simulink model "fft_test"  (Simulink 7.4)
settings: Solver=VariableStepDiscrete  StartTime=0.0  StopTime=500  RelTol=1e-3
libraries: xbsIndex_r4 x1178, casper_library_misc x68, casper_library_delays x13, casper_library_reorder x4, casper_library_ffts_twiddle x2
(part 7 of 11)

== system fft_test/fft/fft_direct/butterfly2_1/twiddle ==
  a : Inport
  b : Inport  Port=2
  sync : Inport  Port=3
  AddSub : xbsIndex_r4/AddSub  mode=Subtraction  use_carryin=off  use_carryout=off  en=off  latency=add_latency  precision=Full  arith_type=Unsigned  n_bits=16  bin_pt=14  quantization=Truncate  overflow=Wrap  dbl_ovrd=off  use_behavioral_HDL=on  hw_selection=Fabric  pipelined=off  block_type=addsub
  AddSub1 : xbsIndex_r4/AddSub  mode=Addition  use_carryin=off  use_carryout=off  en=off  latency=add_latency  precision=Full  arith_type=Unsigned  n_bits=16  bin_pt=14  quantization=Truncate  overflow=Wrap  dbl_ovrd=off  use_behavioral_HDL=on  hw_selection=Fabric  pipelined=off  block_type=addsub
  AddSub2 : xbsIndex_r4/AddSub  mode=Addition  use_carryin=off  use_carryout=off  en=off  latency=add_latency  precision=Full  arith_type=Unsigned  n_bits=16  bin_pt=14  quantization=Truncate  overflow=Wrap  dbl_ovrd=off  use_behavioral_HDL=on  hw_selection=Fabric  pipelined=off  block_type=addsub
  AddSub3 : xbsIndex_r4/AddSub  mode=Subtraction  use_carryin=off  use_carryout=off  en=off  latency=add_latency  precision=Full  arith_type=Unsigned  n_bits=16  bin_pt=14  quantization=Truncate  overflow=Wrap  dbl_ovrd=off  use_behavioral_HDL=on  hw_selection=Fabric  pipelined=off  block_type=addsub
  AddSub4 : xbsIndex_r4/AddSub  mode=Addition  use_carryin=off  use_carryout=off  en=off  latency=add_latency  precision=Full  arith_type=Unsigned  n_bits=16  bin_pt=14  quantization=Truncate  overflow=Wrap  dbl_ovrd=off  use_behavioral_HDL=on  hw_selection=Fabric  pipelined=off  block_type=addsub
  c_to_ri1 : casper_library_misc/c_to_ri  SystemSampleTime=-1  n_bits=8  bin_pt=7
      settings: AttributesFormatString=8_7 r/i
  c_to_ri2 : casper_library_misc/c_to_ri  SystemSampleTime=-1  n_bits=7  bin_pt=5
      settings: AttributesFormatString=7_5 r/i
  c_to_ri3 : casper_library_misc/c_to_ri  SystemSampleTime=-1  n_bits=input_bit_width  bin_pt=input_bit_width-1
      settings: AttributesFormatString=8_7 r/i
  coeff_gen : Subsystem  AncestorBlock=casper_library_ffts_twiddle_coeff_gen/coeff_gen  mask(coeff_gen){Coeffs=getfield( getfield( get_param( gcb,'UserData' ), 'parameters'),'Coeffs'), coeff_bit_width=7, StepPeriod=0, bram_latency=1, coeffs_bram=off}
      mask prompts: Coeffs "Coefficients: (0 to 2^(FFTSize-1)-1)"; coeff_bit_width "Coefficient Bit Width:"; StepPeriod "Step Period: (2^?)"; bram_latency "Latency:"; coeffs_bram "Store coefficients in BRAM"
      mask help: Generates a sequence of complex coefficients
      mask init:
      | coeff_gen_init( gcb, ...
      |     'Coeffs', Coeffs, ...
      |     'coeff_bit_width', coeff_bit_width, ...
      |     'StepPeriod', StepPeriod, ...
      |     'bram_latency', bram_latency, ...
      |     'coeffs_bram', coeffs_bram);
      settings: AttributesFormatString=16 @ (7,5)
      mask CallbackString:
      | Coeffs = eval(get_param(gcb, 'Coeffs'));
      | if( length(Coeffs) == 1 ),
      |     set_param(gcb, 'MaskVisibilities',{'on','on','off','off','off'});
      | else
      |     set_param(gcb, 'MaskVisibilities',{'on','on','on','on','on'});
      | end||||
  convert2 : xbsIndex_r4/Convert  arith_type="Signed  (2's comp)"  n_bits=input_bit_width+5  bin_pt=input_bit_width+1  quantization="Round  (unbiased: +/- Inf)"  overflow=Saturate  latency=conv_latency  dbl_ovrd=off  pipeline=on  block_type=convert
      settings: block_version=11.4
  convert3 : xbsIndex_r4/Convert  arith_type="Signed  (2's comp)"  n_bits=input_bit_width+5  bin_pt=input_bit_width+1  quantization="Round  (unbiased: +/- Inf)"  overflow=Saturate  latency=conv_latency  dbl_ovrd=off  pipeline=on  block_type=convert
      settings: block_version=11.4
  delay0 : xbsIndex_r4/Delay  en=off  latency=mult_latency + 2*add_latency + bram_latency + conv_latency  dbl_ovrd=off  reg_retiming=off  block_type=delay
      settings: block_version=11.4
  delay1 : xbsIndex_r4/Delay  en=off  latency=bram_latency  dbl_ovrd=off  reg_retiming=off  block_type=delay
      settings: block_version=11.4
  delay2 : xbsIndex_r4/Delay  en=off  latency=mult_latency + 2*add_latency + bram_latency + conv_latency  dbl_ovrd=off  reg_retiming=off  block_type=delay
      settings: block_version=11.4
  delay3 : xbsIndex_r4/Delay  en=off  latency=add_latency  dbl_ovrd=off  reg_retiming=on  block_type=delay
      settings: block_version=11.4
  delay4 : xbsIndex_r4/Delay  en=off  latency=add_latency  dbl_ovrd=off  reg_retiming=on  block_type=delay
      settings: block_version=11.4
  delay5 : xbsIndex_r4/Delay  en=off  latency=add_latency  dbl_ovrd=off  reg_retiming=on  block_type=delay
      settings: block_version=11.4
  mult0 : xbsIndex_r4/Mult  precision=Full  arith_type="Signed  (2's comp)"  n_bits=16  bin_pt=14  quantization=Truncate  overflow=Wrap  en=off  latency=mult_latency  dbl_ovrd=off  use_behavioral_HDL=on  opt=Speed  use_embedded=off  optimum_pipeline=off  pipeline=on  use_rpm=on  placement_style=Triangular  block_type=mult
      settings: block_version=11.4
  mult1 : xbsIndex_r4/Mult  precision=Full  arith_type="Signed  (2's comp)"  n_bits=16  bin_pt=14  quantization=Truncate  overflow=Wrap  en=off  latency=mult_latency  dbl_ovrd=off  use_behavioral_HDL=on  opt=Speed  use_embedded=off  optimum_pipeline=off  pipeline=on  use_rpm=on  placement_style=Triangular  block_type=mult
      settings: block_version=11.4
  mult2 : xbsIndex_r4/Mult  precision=Full  arith_type="Signed  (2's comp)"  n_bits=16  bin_pt=14  quantization=Truncate  overflow=Wrap  en=off  latency=mult_latency  dbl_ovrd=off  use_behavioral_HDL=on  opt=Speed  use_embedded=off  optimum_pipeline=off  pipeline=on  use_rpm=on  placement_style=Triangular  block_type=mult
      settings: block_version=11.4
  a_re : Outport
  a_im : Outport  Port=2
  bw_re : Outport  Port=3
  bw_im : Outport  Port=4
  sync_out : Outport  Port=5
  wires:
  a/1 -> delay0/1
  delay0/1 -> c_to_ri1/1
  c_to_ri1/1 -> a_re/1
  c_to_ri1/2 -> a_im/1
  sync/1 -> delay2/1, coeff_gen/1(rst)
  delay2/1 -> sync_out/1
  coeff_gen/1(w) -> c_to_ri2/1
  c_to_ri2/1 -> AddSub2/1, AddSub3/2, delay5/1
  c_to_ri2/2 -> AddSub2/2, AddSub3/1
  b/1 -> delay1/1
  delay1/1 -> c_to_ri3/1
  c_to_ri3/1 -> AddSub1/1, delay3/1
  c_to_ri3/2 -> AddSub1/2, delay4/1
  AddSub1/1 -> mult0/1
  delay5/1 -> mult0/2
  delay4/1 -> mult1/1
  AddSub2/1 -> mult1/2
  delay3/1 -> mult2/1
  AddSub3/1 -> mult2/2
  mult0/1 -> AddSub/1, AddSub4/1
  mult1/1 -> AddSub/2
  mult2/1 -> AddSub4/2
  AddSub/1 -> convert2/1
  convert2/1 -> bw_re/1
  AddSub4/1 -> convert3/1
  convert3/1 -> bw_im/1

== system fft_test/fft/fft_unscrambler/square_transposer/barrel_switcher ==
  sel : Inport  OutDataType=sfix(16)  OutScaling=2^0
  sync_in : Inport  Port=2  OutDataType=sfix(16)  OutScaling=2^0
  In1 : Inport  Port=3  OutDataType=sfix(16)  OutScaling=2^0
  In2 : Inport  Port=4  OutDataType=sfix(16)  OutScaling=2^0
  In3 : Inport  Port=5
  In4 : Inport  Port=6
  Delay1 : xbsIndex_r4/Delay  en=off  latency=1  dbl_ovrd=off  reg_retiming=off  block_type=delay
      settings: block_version=10.1.1
  Delay_sync : xbsIndex_r4/Delay  en=off  latency=2  dbl_ovrd=off  reg_retiming=off  block_type=delay
      settings: xl_area=[0, 0, 0, 0, 0, 0, 0]  block_version=9.1.01
  Mux11 : xbsIndex_r4/Mux  inputs=2  en=off  latency=1  precision=Full  arith_type="Signed  (2's comp)"  n_bits=8  bin_pt=2  quantization=Truncate  overflow=Wrap  dbl_ovrd=off  block_type=mux
      settings: xl_area=[0, 0, 0, 0, 0, 0, 0]  block_version=9.1.01
  Mux{12,22,31..32,41..42} (6 alike) : xbsIndex_r4/Mux  inputs=2  en=off  latency=1  precision=Full  arith_type=Unsigned  n_bits=16  bin_pt=14  quantization=Truncate  overflow=Wrap  dbl_ovrd=off  block_type=mux
      settings: block_version=10.1.1
  Mux21 : xbsIndex_r4/Mux  inputs=2  en=off  latency=1  precision=Full  arith_type="Signed  (2's comp)"  n_bits=8  bin_pt=2  quantization=Truncate  overflow=Wrap  dbl_ovrd=off  block_type=mux
      settings: xl_area=[0, 0, 0, 0, 0, 0, 0]  block_version=9.1.01
  Slice1 : xbsIndex_r4/Slice  nbits=1  boolean_output=off  mode=Upper Bit Location + Width  bit1=-0  base1=MSB of Input  bit0=0  base0=LSB of Input  dbl_ovrd=off  block_type=slice
      settings: infoedit="Extracts a given range of bits from each input sample and presents it at the output.  The output type is ordinarily unsigned with binary point at zero, but can be Boolean when the slice is one bit wide.<P><P>Hardware notes: In hardware this block costs nothing."  block_version=9.1.01
  Slice2 : xbsIndex_r4/Slice  nbits=1  boolean_output=off  mode=Upper Bit Location + Width  bit1=-1  base1=MSB of Input  bit0=0  base0=LSB of Input  dbl_ovrd=off  block_type=slice
      settings: infoedit="Extracts a given range of bits from each input sample and presents it at the output.  The output type is ordinarily unsigned with binary point at zero, but can be Boolean when the slice is one bit wide.<P><P>Hardware notes: In hardware this block costs nothing."  block_version=10.1.1
  sync_out : Outport  OutDataType=sfix(16)  OutScaling=2^0
  Out1 : Outport  Port=2  OutDataType=sfix(16)  OutScaling=2^0
  Out2 : Outport  Port=3  OutDataType=sfix(16)  OutScaling=2^0
  Out3 : Outport  Port=4
  Out4 : Outport  Port=5
  wires:
  sync_in/1 -> Delay_sync/1
  Delay_sync/1 -> sync_out/1
  sel/1 -> Slice1/1, Delay1/1
  Delay1/1 -> Slice2/1
  Slice1/1 -> Mux11/1, Mux21/1, Mux31/1, Mux41/1
  Slice2/1 -> Mux12/1, Mux22/1, Mux32/1, Mux42/1
  In1/1 -> Mux11/2, Mux31/3
  Mux12/1 -> Out1/1
  In2/1 -> Mux21/2, Mux41/3
  Mux22/1 -> Out2/1
  In3/1 -> Mux31/2, Mux11/3
  Mux32/1 -> Out3/1
  In4/1 -> Mux41/2, Mux21/3
  Mux42/1 -> Out4/1
  Mux11/1 -> Mux12/2, Mux42/3
  Mux21/1 -> Mux22/2, Mux12/3
  Mux31/1 -> Mux32/2, Mux22/3
  Mux41/1 -> Mux42/2, Mux32/3

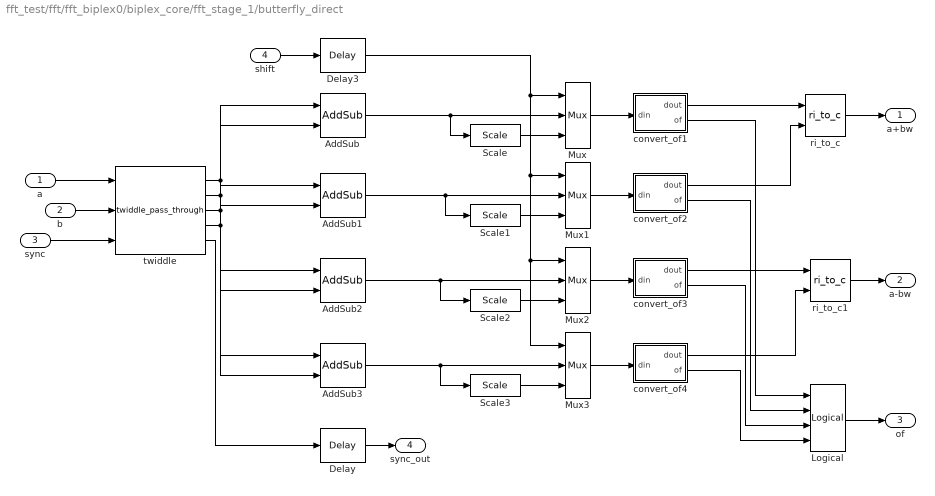
== system fft_test/fft/fft_biplex0/biplex_core/fft_stage_1/butterfly_direct ==
  a : Inport  OutDataType=sfix(16)  OutScaling=2^0
  b : Inport  Port=2  OutDataType=sfix(16)  OutScaling=2^0
  sync : Inport  Port=3  OutDataType=sfix(16)  OutScaling=2^0
  shift : Inport  Port=4  OutDataType=sfix(16)  OutScaling=2^0
  AddSub : xbsIndex_r4/AddSub  mode=Addition  use_carryin=off  use_carryout=off  en=off  latency=add_latency  precision=Full  arith_type=Unsigned  n_bits=8  bin_pt=2  quantization=Truncate  overflow=Wrap  dbl_ovrd=off  use_behavioral_HDL=off  hw_selection=DSP48  pipelined=on  use_rpm=on  block_type=addsub
      settings: xl_area=[0, 0, 0, 0, 0, 0, 0]  block_version=9.1.01
  AddSub1 : xbsIndex_r4/AddSub  mode=Addition  use_carryin=off  use_carryout=off  en=off  latency=add_latency  precision=Full  arith_type=Unsigned  n_bits=8  bin_pt=2  quantization=Truncate  overflow=Wrap  dbl_ovrd=off  use_behavioral_HDL=off  hw_selection=DSP48  pipelined=on  use_rpm=on  block_type=addsub
      settings: xl_area=[0, 0, 0, 0, 0, 0, 0]  block_version=9.1.01
  AddSub2 : xbsIndex_r4/AddSub  mode=Subtraction  use_carryin=off  use_carryout=off  en=off  latency=add_latency  precision=Full  arith_type=Unsigned  n_bits=8  bin_pt=2  quantization=Truncate  overflow=Wrap  dbl_ovrd=off  use_behavioral_HDL=off  hw_selection=DSP48  pipelined=on  use_rpm=on  block_type=addsub
      settings: xl_area=[0, 0, 0, 0, 0, 0, 0]  block_version=9.1.01
  AddSub3 : xbsIndex_r4/AddSub  mode=Subtraction  use_carryin=off  use_carryout=off  en=off  latency=add_latency  precision=Full  arith_type=Unsigned  n_bits=8  bin_pt=2  quantization=Truncate  overflow=Wrap  dbl_ovrd=off  use_behavioral_HDL=off  hw_selection=DSP48  pipelined=on  use_rpm=on  block_type=addsub
      settings: xl_area=[0, 0, 0, 0, 0, 0, 0]  block_version=9.1.01
  Delay : xbsIndex_r4/Delay  en=off  latency=add_latency + conv_latency + 1  dbl_ovrd=off  reg_retiming=on  block_type=delay
      settings: xl_area=[0, 0, 0, 0, 0, 0, 0]  block_version=9.1.01
  Delay3 : xbsIndex_r4/Delay  en=off  latency=add_latency  dbl_ovrd=off  reg_retiming=off  block_type=delay
      settings: xl_area=[0, 0, 0, 0, 0, 0, 0]  block_version=9.1.01
  Logical : xbsIndex_r4/Logical  logical_function=OR  inputs=4  en=off  latency=0  precision=Full  arith_type=Unsigned  n_bits=16  bin_pt=0  align_bp=on  dbl_ovrd=off  block_type=logical
      settings: block_version=10.1.1
  Mux{,1..3} (4 alike) : xbsIndex_r4/Mux  inputs=2  en=off  latency=1  precision=Full  arith_type="Signed  (2's comp)"  n_bits=8  bin_pt=2  quantization=Truncate  overflow=Wrap  dbl_ovrd=off  block_type=mux
      settings: xl_area=[0, 0, 0, 0, 0, 0, 0]  block_version=9.1.01
  Scale{,1..3} (4 alike) : xbsIndex_r4/Scale  scale_factor=-1  dbl_ovrd=off  block_type=scale
      settings: infoedit=Scales input by a power of two by adjusting the binary point position.<P><P>Hardware notes: In hardware this block costs nothing.  block_version=9.1.01
  convert_of1 : Subsystem  AncestorBlock=casper_library_misc/convert_of  mask(convert_of){bit_width_i=10, binary_point_i=8, bit_width_o=8, binary_point_o=7, latency=2, overflow=Saturate, quantization=Round  (unbiased: +/- Inf)}
      mask prompts: bit_width_i "Bit Width In"; binary_point_i "Binary Point In"; bit_width_o "Bit Width Out"; binary_point_o "Binary Point Out"; overflow "Overflow Behaviour"; quantization "Quantization Behaviour"
      mask help:
      | Converts from one 2's complement bit-width
      | and/or binary point position to another.
      | Includes underflow/overflow indicator.
      mask init: same as fft_test/fft/fft_direct/butterfly1_0/convert_of1
      settings: AttributesFormatString=[10,8]->[8,7]
      mask StyleString: edit,edit,edit,edit,edit,popup(Wrap|Saturate|Error),popup(Truncate|Round  (unbiased: +/- Inf)|Round  (unbiased: even values))
  convert_of2 : Subsystem  AncestorBlock=casper_library_misc/convert_of  mask(convert_of){bit_width_i=10, binary_point_i=8, bit_width_o=8, binary_point_o=7, latency=2, overflow=Saturate, quantization=Round  (unbiased: +/- Inf)}
      mask prompts: bit_width_i "Bit Width In"; binary_point_i "Binary Point In"; bit_width_o "Bit Width Out"; binary_point_o "Binary Point Out"; overflow "Overflow Behaviour"; quantization "Quantization Behaviour"
      mask help:
      | Converts from one 2's complement bit-width
      | and/or binary point position to another.
      | Includes underflow/overflow indicator.
      mask init: same as fft_test/fft/fft_direct/butterfly1_0/convert_of1
      settings: AttributesFormatString=[10,8]->[8,7]
      mask StyleString: edit,edit,edit,edit,edit,popup(Wrap|Saturate|Error),popup(Truncate|Round  (unbiased: +/- Inf)|Round  (unbiased: even values))
  convert_of3 : Subsystem  AncestorBlock=casper_library_misc/convert_of  mask(convert_of){bit_width_i=10, binary_point_i=8, bit_width_o=8, binary_point_o=7, latency=2, overflow=Saturate, quantization=Round  (unbiased: +/- Inf)}
      mask prompts: bit_width_i "Bit Width In"; binary_point_i "Binary Point In"; bit_width_o "Bit Width Out"; binary_point_o "Binary Point Out"; overflow "Overflow Behaviour"; quantization "Quantization Behaviour"
      mask help:
      | Converts from one 2's complement bit-width
      | and/or binary point position to another.
      | Includes underflow/overflow indicator.
      mask init: same as fft_test/fft/fft_direct/butterfly1_0/convert_of1
      settings: AttributesFormatString=[10,8]->[8,7]
      mask StyleString: edit,edit,edit,edit,edit,popup(Wrap|Saturate|Error),popup(Truncate|Round  (unbiased: +/- Inf)|Round  (unbiased: even values))
  convert_of4 : Subsystem  AncestorBlock=casper_library_misc/convert_of  mask(convert_of){bit_width_i=10, binary_point_i=8, bit_width_o=8, binary_point_o=7, latency=2, overflow=Saturate, quantization=Round  (unbiased: +/- Inf)}
      mask prompts: bit_width_i "Bit Width In"; binary_point_i "Binary Point In"; bit_width_o "Bit Width Out"; binary_point_o "Binary Point Out"; overflow "Overflow Behaviour"; quantization "Quantization Behaviour"
      mask help:
      | Converts from one 2's complement bit-width
      | and/or binary point position to another.
      | Includes underflow/overflow indicator.
      mask init: same as fft_test/fft/fft_direct/butterfly1_0/convert_of1
      settings: AttributesFormatString=[10,8]->[8,7]
      mask StyleString: edit,edit,edit,edit,edit,popup(Wrap|Saturate|Error),popup(Truncate|Round  (unbiased: +/- Inf)|Round  (unbiased: even values))
  ri_to_c : casper_library_misc/ri_to_c  SystemSampleTime=-1
  ri_to_c1 : casper_library_misc/ri_to_c  SystemSampleTime=-1
  twiddle : casper_library_ffts_twiddle/twiddle_pass_through  SystemSampleTime=-1  FFTSize=4  input_bit_width=8  add_latency=2  mult_latency=3  bram_latency=1  conv_latency=2  opt_target=multipliers
  a+bw : Outport  OutDataType=sfix(16)  OutScaling=2^0
  a-bw : Outport  Port=2  OutDataType=sfix(16)  OutScaling=2^0
  of : Outport  Port=3  OutDataType=sfix(16)  OutScaling=2^0
  sync_out : Outport  Port=4  OutDataType=sfix(16)  OutScaling=2^0
  wires:
  convert_of4/2(of) -> Logical/4
  convert_of3/2(of) -> Logical/3
  convert_of2/2(of) -> Logical/2
  convert_of1/2(of) -> Logical/1
  convert_of4/1(dout) -> ri_to_c1/2
  Mux3/1 -> convert_of4/1(din)
  AddSub3/1 -> Scale3/1, Mux3/2
  Scale3/1 -> Mux3/3
  convert_of3/1(dout) -> ri_to_c1/1
  Mux2/1 -> convert_of3/1(din)
  AddSub2/1 -> Scale2/1, Mux2/2
  Scale2/1 -> Mux2/3
  convert_of2/1(dout) -> ri_to_c/2
  Mux1/1 -> convert_of2/1(din)
  AddSub1/1 -> Scale1/1, Mux1/2
  Scale1/1 -> Mux1/3
  convert_of1/1(dout) -> ri_to_c/1
  Mux/1 -> convert_of1/1(din)
  twiddle/4 -> AddSub3/2, AddSub1/2
  twiddle/3 -> AddSub2/2, AddSub/2
  twiddle/2 -> AddSub3/1, AddSub1/1
  twiddle/1 -> AddSub2/1, AddSub/1
  sync/1 -> twiddle/3
  b/1 -> twiddle/2
  a/1 -> twiddle/1
  ri_to_c/1 -> a+bw/1
  ri_to_c1/1 -> a-bw/1
  Delay/1 -> sync_out/1
  AddSub/1 -> Mux/2, Scale/1
  shift/1 -> Delay3/1
  Scale/1 -> Mux/3
  Delay3/1 -> Mux3/1, Mux2/1, Mux1/1, Mux/1
  Logical/1 -> of/1
  twiddle/5 -> Delay/1

== system fft_test/fft/fft_biplex0/biplex_core/fft_stage_1/delay_b ==
  In1 : Inport  OutDataType=sfix(16)  OutScaling=2^0
  delay_slr : xbsIndex_r4/Delay  en=off  latency=DelayLen  dbl_ovrd=off  reg_retiming=off  block_type=delay
      settings: xl_area=[0, 0, 0, 0, 0, 0, 0]  block_version=9.1.01
  Out1 : Outport  OutDataType=sfix(16)  OutScaling=2^0
  wires:
  delay_slr/1 -> Out1/1
  In1/1 -> delay_slr/1

== system fft_test/fft/fft_biplex0/biplex_core/fft_stage_1/delay_f ==
  In1 : Inport  OutDataType=sfix(16)  OutScaling=2^0
  delay_slr : xbsIndex_r4/Delay  en=off  latency=DelayLen  dbl_ovrd=off  reg_retiming=off  block_type=delay
      settings: xl_area=[0, 0, 0, 0, 0, 0, 0]  block_version=9.1.01
  Out1 : Outport  OutDataType=sfix(16)  OutScaling=2^0
  wires:
  delay_slr/1 -> Out1/1
  In1/1 -> delay_slr/1

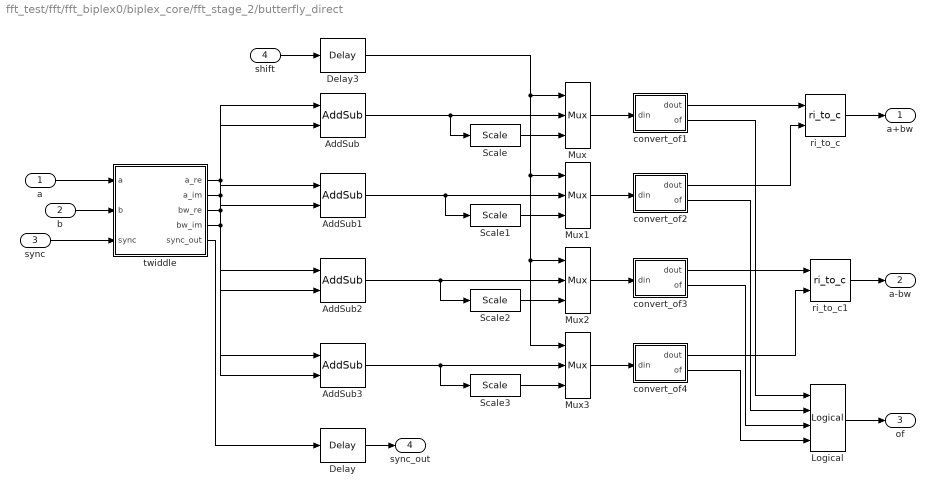
== system fft_test/fft/fft_biplex0/biplex_core/fft_stage_2/butterfly_direct ==
  a : Inport  OutDataType=sfix(16)  OutScaling=2^0
  b : Inport  Port=2  OutDataType=sfix(16)  OutScaling=2^0
  sync : Inport  Port=3  OutDataType=sfix(16)  OutScaling=2^0
  shift : Inport  Port=4  OutDataType=sfix(16)  OutScaling=2^0
  AddSub : xbsIndex_r4/AddSub  mode=Addition  use_carryin=off  use_carryout=off  en=off  latency=add_latency  precision=Full  arith_type=Unsigned  n_bits=8  bin_pt=2  quantization=Truncate  overflow=Wrap  dbl_ovrd=off  use_behavioral_HDL=off  hw_selection=DSP48  pipelined=on  use_rpm=on  block_type=addsub
      settings: xl_area=[0, 0, 0, 0, 0, 0, 0]  block_version=9.1.01
  AddSub1 : xbsIndex_r4/AddSub  mode=Addition  use_carryin=off  use_carryout=off  en=off  latency=add_latency  precision=Full  arith_type=Unsigned  n_bits=8  bin_pt=2  quantization=Truncate  overflow=Wrap  dbl_ovrd=off  use_behavioral_HDL=off  hw_selection=DSP48  pipelined=on  use_rpm=on  block_type=addsub
      settings: xl_area=[0, 0, 0, 0, 0, 0, 0]  block_version=9.1.01
  AddSub2 : xbsIndex_r4/AddSub  mode=Subtraction  use_carryin=off  use_carryout=off  en=off  latency=add_latency  precision=Full  arith_type=Unsigned  n_bits=8  bin_pt=2  quantization=Truncate  overflow=Wrap  dbl_ovrd=off  use_behavioral_HDL=off  hw_selection=DSP48  pipelined=on  use_rpm=on  block_type=addsub
      settings: xl_area=[0, 0, 0, 0, 0, 0, 0]  block_version=9.1.01
  AddSub3 : xbsIndex_r4/AddSub  mode=Subtraction  use_carryin=off  use_carryout=off  en=off  latency=add_latency  precision=Full  arith_type=Unsigned  n_bits=8  bin_pt=2  quantization=Truncate  overflow=Wrap  dbl_ovrd=off  use_behavioral_HDL=off  hw_selection=DSP48  pipelined=on  use_rpm=on  block_type=addsub
      settings: xl_area=[0, 0, 0, 0, 0, 0, 0]  block_version=9.1.01
  Delay : xbsIndex_r4/Delay  en=off  latency=add_latency + conv_latency + 1  dbl_ovrd=off  reg_retiming=on  block_type=delay
      settings: xl_area=[0, 0, 0, 0, 0, 0, 0]  block_version=9.1.01
  Delay3 : xbsIndex_r4/Delay  en=off  latency=add_latency  dbl_ovrd=off  reg_retiming=off  block_type=delay
      settings: xl_area=[0, 0, 0, 0, 0, 0, 0]  block_version=9.1.01
  Logical : xbsIndex_r4/Logical  logical_function=OR  inputs=4  en=off  latency=0  precision=Full  arith_type=Unsigned  n_bits=16  bin_pt=0  align_bp=on  dbl_ovrd=off  block_type=logical
      settings: block_version=10.1.1
  Mux{,1..3} (4 alike) : xbsIndex_r4/Mux  inputs=2  en=off  latency=1  precision=Full  arith_type="Signed  (2's comp)"  n_bits=8  bin_pt=2  quantization=Truncate  overflow=Wrap  dbl_ovrd=off  block_type=mux
      settings: xl_area=[0, 0, 0, 0, 0, 0, 0]  block_version=9.1.01
  Scale{,1..3} (4 alike) : xbsIndex_r4/Scale  scale_factor=-1  dbl_ovrd=off  block_type=scale
      settings: infoedit=Scales input by a power of two by adjusting the binary point position.<P><P>Hardware notes: In hardware this block costs nothing.  block_version=9.1.01
  convert_of1 : Subsystem  AncestorBlock=casper_library_misc/convert_of  mask(convert_of){bit_width_i=10, binary_point_i=8, bit_width_o=8, binary_point_o=7, latency=2, overflow=Saturate, quantization=Round  (unbiased: +/- Inf)}
      mask prompts: bit_width_i "Bit Width In"; binary_point_i "Binary Point In"; bit_width_o "Bit Width Out"; binary_point_o "Binary Point Out"; overflow "Overflow Behaviour"; quantization "Quantization Behaviour"
      mask help:
      | Converts from one 2's complement bit-width
      | and/or binary point position to another.
      | Includes underflow/overflow indicator.
      mask init: same as fft_test/fft/fft_direct/butterfly1_0/convert_of1
      settings: AttributesFormatString=[10,8]->[8,7]
      mask StyleString: edit,edit,edit,edit,edit,popup(Wrap|Saturate|Error),popup(Truncate|Round  (unbiased: +/- Inf)|Round  (unbiased: even values))
  convert_of2 : Subsystem  AncestorBlock=casper_library_misc/convert_of  mask(convert_of){bit_width_i=10, binary_point_i=8, bit_width_o=8, binary_point_o=7, latency=2, overflow=Saturate, quantization=Round  (unbiased: +/- Inf)}
      mask prompts: bit_width_i "Bit Width In"; binary_point_i "Binary Point In"; bit_width_o "Bit Width Out"; binary_point_o "Binary Point Out"; overflow "Overflow Behaviour"; quantization "Quantization Behaviour"
      mask help:
      | Converts from one 2's complement bit-width
      | and/or binary point position to another.
      | Includes underflow/overflow indicator.
      mask init: same as fft_test/fft/fft_direct/butterfly1_0/convert_of1
      settings: AttributesFormatString=[10,8]->[8,7]
      mask StyleString: edit,edit,edit,edit,edit,popup(Wrap|Saturate|Error),popup(Truncate|Round  (unbiased: +/- Inf)|Round  (unbiased: even values))
  convert_of3 : Subsystem  AncestorBlock=casper_library_misc/convert_of  mask(convert_of){bit_width_i=10, binary_point_i=8, bit_width_o=8, binary_point_o=7, latency=2, overflow=Saturate, quantization=Round  (unbiased: +/- Inf)}
      mask prompts: bit_width_i "Bit Width In"; binary_point_i "Binary Point In"; bit_width_o "Bit Width Out"; binary_point_o "Binary Point Out"; overflow "Overflow Behaviour"; quantization "Quantization Behaviour"
      mask help:
      | Converts from one 2's complement bit-width
      | and/or binary point position to another.
      | Includes underflow/overflow indicator.
      mask init: same as fft_test/fft/fft_direct/butterfly1_0/convert_of1
      settings: AttributesFormatString=[10,8]->[8,7]
      mask StyleString: edit,edit,edit,edit,edit,popup(Wrap|Saturate|Error),popup(Truncate|Round  (unbiased: +/- Inf)|Round  (unbiased: even values))
  convert_of4 : Subsystem  AncestorBlock=casper_library_misc/convert_of  mask(convert_of){bit_width_i=10, binary_point_i=8, bit_width_o=8, binary_point_o=7, latency=2, overflow=Saturate, quantization=Round  (unbiased: +/- Inf)}
      mask prompts: bit_width_i "Bit Width In"; binary_point_i "Binary Point In"; bit_width_o "Bit Width Out"; binary_point_o "Binary Point Out"; overflow "Overflow Behaviour"; quantization "Quantization Behaviour"
      mask help:
      | Converts from one 2's complement bit-width
      | and/or binary point position to another.
      | Includes underflow/overflow indicator.
      mask init: same as fft_test/fft/fft_direct/butterfly1_0/convert_of1
      settings: AttributesFormatString=[10,8]->[8,7]
      mask StyleString: edit,edit,edit,edit,edit,popup(Wrap|Saturate|Error),popup(Truncate|Round  (unbiased: +/- Inf)|Round  (unbiased: even values))
  ri_to_c : casper_library_misc/ri_to_c  SystemSampleTime=-1
  ri_to_c1 : casper_library_misc/ri_to_c  SystemSampleTime=-1
  twiddle : Subsystem  AncestorBlock=casper_library_ffts_twiddle/twiddle_stage_2  mask(twiddle_pass_through){FFTSize=4, input_bit_width=8, add_latency=2, mult_latency=3, bram_latency=1, conv_latency=2, opt_target=multipliers}
      mask prompts: FFTSize "FFT Size (2^?)"; input_bit_width "Input Bit Width"; add_latency "Add Latency"; mult_latency "Mult Latency"; bram_latency "BRAM Latency"; conv_latency "Convert latency"; opt_target "Use less"
      mask help:
      | Used in FFT library. Used when coefficients
      | are 2^0 i.e just pass data through without delays
      mask init:
      | set_param(gcb,'LinkStatus','inactive');
      | if(strcmp(opt_target, 'logic')), 
      |     lat = add_latency;
      |     lat_str = 'add_latency';
      | else,
      |     lat = add_latency*2;
      |     lat_str = 'add_latency*2';
      | end
      | set_param([gcb,'/delay0'], 'latency', ...
      |     ['bram_latency+mult_latency+conv_latency+',lat_str]);
      | set_param([gcb,'/delay1'], 'latency', ...
      |     ['bram_latency+mult_latency+conv_latency+',lat_str]);
      | set_param([gcb,'/mux0'], 'latency', ...
      |     num2str(mult_latency+conv_latency+lat));
      | set_param([gcb,'/mux1'], 'latency', ...
      |     num2str(mult_latency+conv_latency+lat));
      | set_param([gcb,'/delay6'], 'latency', ...
      |     ['mult_latency+conv_latency+',lat_str]);
      mask StyleString: edit,edit,edit,edit,edit,edit,popup(logic|multipliers)
  a+bw : Outport  OutDataType=sfix(16)  OutScaling=2^0
  a-bw : Outport  Port=2  OutDataType=sfix(16)  OutScaling=2^0
  of : Outport  Port=3  OutDataType=sfix(16)  OutScaling=2^0
  sync_out : Outport  Port=4  OutDataType=sfix(16)  OutScaling=2^0
  wires:
  convert_of4/2(of) -> Logical/4
  convert_of3/2(of) -> Logical/3
  convert_of2/2(of) -> Logical/2
  convert_of1/2(of) -> Logical/1
  convert_of4/1(dout) -> ri_to_c1/2
  Mux3/1 -> convert_of4/1(din)
  AddSub3/1 -> Scale3/1, Mux3/2
  Scale3/1 -> Mux3/3
  convert_of3/1(dout) -> ri_to_c1/1
  Mux2/1 -> convert_of3/1(din)
  AddSub2/1 -> Scale2/1, Mux2/2
  Scale2/1 -> Mux2/3
  convert_of2/1(dout) -> ri_to_c/2
  Mux1/1 -> convert_of2/1(din)
  AddSub1/1 -> Scale1/1, Mux1/2
  Scale1/1 -> Mux1/3
  convert_of1/1(dout) -> ri_to_c/1
  Mux/1 -> convert_of1/1(din)
  twiddle/4(bw_im) -> AddSub3/2, AddSub1/2
  twiddle/3(bw_re) -> AddSub2/2, AddSub/2
  twiddle/2(a_im) -> AddSub3/1, AddSub1/1
  twiddle/1(a_re) -> AddSub2/1, AddSub/1
  sync/1 -> twiddle/3(sync)
  b/1 -> twiddle/2(b)
  a/1 -> twiddle/1(a)
  ri_to_c/1 -> a+bw/1
  ri_to_c1/1 -> a-bw/1
  Delay/1 -> sync_out/1
  AddSub/1 -> Mux/2, Scale/1
  shift/1 -> Delay3/1
  Scale/1 -> Mux/3
  Delay3/1 -> Mux3/1, Mux2/1, Mux1/1, Mux/1
  Logical/1 -> of/1
  twiddle/5(sync_out) -> Delay/1

== system fft_test/fft/fft_biplex0/biplex_core/fft_stage_2/delay_b ==
  In1 : Inport  OutDataType=sfix(16)  OutScaling=2^0
  delay_slr : xbsIndex_r4/Delay  en=off  latency=DelayLen  dbl_ovrd=off  reg_retiming=off  block_type=delay
      settings: xl_area=[0, 0, 0, 0, 0, 0, 0]  block_version=9.1.01
  Out1 : Outport  OutDataType=sfix(16)  OutScaling=2^0
  wires:
  delay_slr/1 -> Out1/1
  In1/1 -> delay_slr/1

== system fft_test/fft/fft_biplex0/biplex_core/fft_stage_2/delay_f ==
  In1 : Inport  OutDataType=sfix(16)  OutScaling=2^0
  delay_slr : xbsIndex_r4/Delay  en=off  latency=DelayLen  dbl_ovrd=off  reg_retiming=off  block_type=delay
      settings: xl_area=[0, 0, 0, 0, 0, 0, 0]  block_version=9.1.01
  Out1 : Outport  OutDataType=sfix(16)  OutScaling=2^0
  wires:
  delay_slr/1 -> Out1/1
  In1/1 -> delay_slr/1

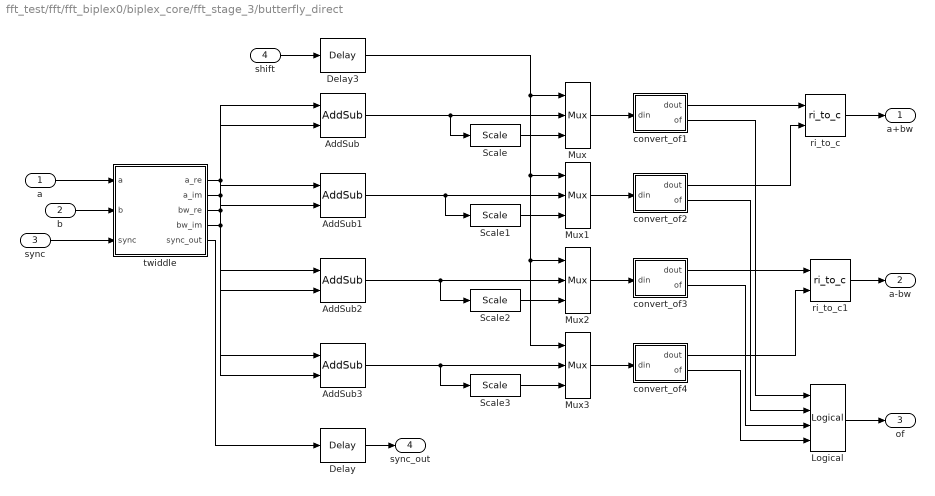
== system fft_test/fft/fft_biplex0/biplex_core/fft_stage_3/butterfly_direct ==
  a : Inport  OutDataType=sfix(16)  OutScaling=2^0
  b : Inport  Port=2  OutDataType=sfix(16)  OutScaling=2^0
  sync : Inport  Port=3  OutDataType=sfix(16)  OutScaling=2^0
  shift : Inport  Port=4  OutDataType=sfix(16)  OutScaling=2^0
  AddSub : xbsIndex_r4/AddSub  mode=Addition  use_carryin=off  use_carryout=off  en=off  latency=add_latency  precision=Full  arith_type=Unsigned  n_bits=8  bin_pt=2  quantization=Truncate  overflow=Wrap  dbl_ovrd=off  use_behavioral_HDL=off  hw_selection=DSP48  pipelined=on  use_rpm=on  block_type=addsub
      settings: xl_area=[0, 0, 0, 0, 0, 0, 0]  block_version=9.1.01
  AddSub1 : xbsIndex_r4/AddSub  mode=Addition  use_carryin=off  use_carryout=off  en=off  latency=add_latency  precision=Full  arith_type=Unsigned  n_bits=8  bin_pt=2  quantization=Truncate  overflow=Wrap  dbl_ovrd=off  use_behavioral_HDL=off  hw_selection=DSP48  pipelined=on  use_rpm=on  block_type=addsub
      settings: xl_area=[0, 0, 0, 0, 0, 0, 0]  block_version=9.1.01
  AddSub2 : xbsIndex_r4/AddSub  mode=Subtraction  use_carryin=off  use_carryout=off  en=off  latency=add_latency  precision=Full  arith_type=Unsigned  n_bits=8  bin_pt=2  quantization=Truncate  overflow=Wrap  dbl_ovrd=off  use_behavioral_HDL=off  hw_selection=DSP48  pipelined=on  use_rpm=on  block_type=addsub
      settings: xl_area=[0, 0, 0, 0, 0, 0, 0]  block_version=9.1.01
  AddSub3 : xbsIndex_r4/AddSub  mode=Subtraction  use_carryin=off  use_carryout=off  en=off  latency=add_latency  precision=Full  arith_type=Unsigned  n_bits=8  bin_pt=2  quantization=Truncate  overflow=Wrap  dbl_ovrd=off  use_behavioral_HDL=off  hw_selection=DSP48  pipelined=on  use_rpm=on  block_type=addsub
      settings: xl_area=[0, 0, 0, 0, 0, 0, 0]  block_version=9.1.01
  Delay : xbsIndex_r4/Delay  en=off  latency=add_latency + conv_latency + 1  dbl_ovrd=off  reg_retiming=on  block_type=delay
      settings: xl_area=[0, 0, 0, 0, 0, 0, 0]  block_version=9.1.01
  Delay3 : xbsIndex_r4/Delay  en=off  latency=add_latency  dbl_ovrd=off  reg_retiming=off  block_type=delay
      settings: xl_area=[0, 0, 0, 0, 0, 0, 0]  block_version=9.1.01
  Logical : xbsIndex_r4/Logical  logical_function=OR  inputs=4  en=off  latency=0  precision=Full  arith_type=Unsigned  n_bits=16  bin_pt=0  align_bp=on  dbl_ovrd=off  block_type=logical
      settings: block_version=10.1.1
  Mux{,1..3} (4 alike) : xbsIndex_r4/Mux  inputs=2  en=off  latency=1  precision=Full  arith_type="Signed  (2's comp)"  n_bits=8  bin_pt=2  quantization=Truncate  overflow=Wrap  dbl_ovrd=off  block_type=mux
      settings: xl_area=[0, 0, 0, 0, 0, 0, 0]  block_version=9.1.01
  Scale{,1..3} (4 alike) : xbsIndex_r4/Scale  scale_factor=-1  dbl_ovrd=off  block_type=scale
      settings: infoedit=Scales input by a power of two by adjusting the binary point position.<P><P>Hardware notes: In hardware this block costs nothing.  block_version=9.1.01
  convert_of1 : Subsystem  AncestorBlock=casper_library_misc/convert_of  mask(convert_of){bit_width_i=15, binary_point_i=10, bit_width_o=8, binary_point_o=7, latency=2, overflow=Saturate, quantization=Round  (unbiased: +/- Inf)}
      mask prompts: bit_width_i "Bit Width In"; binary_point_i "Binary Point In"; bit_width_o "Bit Width Out"; binary_point_o "Binary Point Out"; overflow "Overflow Behaviour"; quantization "Quantization Behaviour"
      mask help:
      | Converts from one 2's complement bit-width
      | and/or binary point position to another.
      | Includes underflow/overflow indicator.
      mask init: same as fft_test/fft/fft_direct/butterfly1_0/convert_of1
      settings: AttributesFormatString=[15,10]->[8,7]
      mask StyleString: edit,edit,edit,edit,edit,popup(Wrap|Saturate|Error),popup(Truncate|Round  (unbiased: +/- Inf)|Round  (unbiased: even values))
  convert_of2 : Subsystem  AncestorBlock=casper_library_misc/convert_of  mask(convert_of){bit_width_i=15, binary_point_i=10, bit_width_o=8, binary_point_o=7, latency=2, overflow=Saturate, quantization=Round  (unbiased: +/- Inf)}
      mask prompts: bit_width_i "Bit Width In"; binary_point_i "Binary Point In"; bit_width_o "Bit Width Out"; binary_point_o "Binary Point Out"; overflow "Overflow Behaviour"; quantization "Quantization Behaviour"
      mask help:
      | Converts from one 2's complement bit-width
      | and/or binary point position to another.
      | Includes underflow/overflow indicator.
      mask init: same as fft_test/fft/fft_direct/butterfly1_0/convert_of1
      settings: AttributesFormatString=[15,10]->[8,7]
      mask StyleString: edit,edit,edit,edit,edit,popup(Wrap|Saturate|Error),popup(Truncate|Round  (unbiased: +/- Inf)|Round  (unbiased: even values))
  convert_of3 : Subsystem  AncestorBlock=casper_library_misc/convert_of  mask(convert_of){bit_width_i=15, binary_point_i=10, bit_width_o=8, binary_point_o=7, latency=2, overflow=Saturate, quantization=Round  (unbiased: +/- Inf)}
      mask prompts: bit_width_i "Bit Width In"; binary_point_i "Binary Point In"; bit_width_o "Bit Width Out"; binary_point_o "Binary Point Out"; overflow "Overflow Behaviour"; quantization "Quantization Behaviour"
      mask help:
      | Converts from one 2's complement bit-width
      | and/or binary point position to another.
      | Includes underflow/overflow indicator.
      mask init: same as fft_test/fft/fft_direct/butterfly1_0/convert_of1
      settings: AttributesFormatString=[15,10]->[8,7]
      mask StyleString: edit,edit,edit,edit,edit,popup(Wrap|Saturate|Error),popup(Truncate|Round  (unbiased: +/- Inf)|Round  (unbiased: even values))
  convert_of4 : Subsystem  AncestorBlock=casper_library_misc/convert_of  mask(convert_of){bit_width_i=15, binary_point_i=10, bit_width_o=8, binary_point_o=7, latency=2, overflow=Saturate, quantization=Round  (unbiased: +/- Inf)}
      mask prompts: bit_width_i "Bit Width In"; binary_point_i "Binary Point In"; bit_width_o "Bit Width Out"; binary_point_o "Binary Point Out"; overflow "Overflow Behaviour"; quantization "Quantization Behaviour"
      mask help:
      | Converts from one 2's complement bit-width
      | and/or binary point position to another.
      | Includes underflow/overflow indicator.
      mask init: same as fft_test/fft/fft_direct/butterfly1_0/convert_of1
      settings: AttributesFormatString=[15,10]->[8,7]
      mask StyleString: edit,edit,edit,edit,edit,popup(Wrap|Saturate|Error),popup(Truncate|Round  (unbiased: +/- Inf)|Round  (unbiased: even values))
  ri_to_c : casper_library_misc/ri_to_c  SystemSampleTime=-1
  ri_to_c1 : casper_library_misc/ri_to_c  SystemSampleTime=-1
  twiddle : Subsystem  AncestorBlock=casper_library_ffts_twiddle/twiddle_general_3mult  mask(twiddle_general_3mult){Coeffs=getfield( getfield( get_param( gcb,'UserData' ), 'parameters'),'Coeffs'), StepPeriod=1, coeffs_bram=off, coeff_bit_width=8, input_bit_width=8, add_latency=2, mult_latency=3, bram_latency=1, conv_latency=2, arch=Virtex5, use_hdl=on, use_embedded=off, quantization=Round  (unbiased: +/- Inf), overflow=Saturate}
      mask prompts: Coeffs "Coefficients:"; StepPeriod "Coefficient Step Period (2^?)"; coeffs_bram "Store coefficients in BRAM"; coeff_bit_width "Coefficient Bit Width"; input_bit_width "Input Bit Width"; add_latency "Add Latency"; mult_latency "Mult Latency"; bram_latency "BRAM Latency"; conv_latency "Convert latency"; arch "Architecture"; use_hdl "Use behavioral HDL for multlipliers"; use_embedded "Use embedded multipliers"; quantization "Quantization Behavior"; overflow "Overflow Behavior"
      mask help:
      | Used in biplex pipelined FFT. Takes advantage that
      | (a+bi)(c+di)=(c(a+b)-b(c+d))+i(b(c+d)+a(c-d)) to
      | save on multipliers at expense of adders.
      mask init: same as fft_test/fft/fft_direct/butterfly1_0/twiddle
      settings: AttributesFormatString=|
      | data=(8,7)
      | coeffs=(7,5)
      | Virtex5
      | (Round  (unbiased: +/- Inf),Saturate)
      mask StyleString: edit,edit,checkbox,edit,edit,edit,edit,edit,edit,popup(Virtex2Pro|Virtex5),checkbox,checkbox,popup(Truncate|Round  (unbiased: +/- Inf)|Round  (unbiased: Even Values)),popup(Wrap|Saturate|Error)
      mask CallbackString:
      | ||||||||||use_hdl = get_param(gcb,'use_hdl');
      | visibs = get_param(gcb, 'MaskVisibilities');
      | if( strcmp(use_hdl,'on')),
      |     set_param(gcb, 'use_embedded','off');
      |     visibs{12} = 'off';
      | else,
      |     visibs{12} = 'on';
      | end
      | set_param(gcb, 'MaskVisibilities', visibs);
      | |||
  a+bw : Outport  OutDataType=sfix(16)  OutScaling=2^0
  a-bw : Outport  Port=2  OutDataType=sfix(16)  OutScaling=2^0
  of : Outport  Port=3  OutDataType=sfix(16)  OutScaling=2^0
  sync_out : Outport  Port=4  OutDataType=sfix(16)  OutScaling=2^0
  wires:
  convert_of4/2(of) -> Logical/4
  convert_of3/2(of) -> Logical/3
  convert_of2/2(of) -> Logical/2
  convert_of1/2(of) -> Logical/1
  convert_of4/1(dout) -> ri_to_c1/2
  Mux3/1 -> convert_of4/1(din)
  AddSub3/1 -> Scale3/1, Mux3/2
  Scale3/1 -> Mux3/3
  convert_of3/1(dout) -> ri_to_c1/1
  Mux2/1 -> convert_of3/1(din)
  AddSub2/1 -> Scale2/1, Mux2/2
  Scale2/1 -> Mux2/3
  convert_of2/1(dout) -> ri_to_c/2
  Mux1/1 -> convert_of2/1(din)
  AddSub1/1 -> Scale1/1, Mux1/2
  Scale1/1 -> Mux1/3
  convert_of1/1(dout) -> ri_to_c/1
  Mux/1 -> convert_of1/1(din)
  twiddle/4(bw_im) -> AddSub3/2, AddSub1/2
  twiddle/3(bw_re) -> AddSub2/2, AddSub/2
  twiddle/2(a_im) -> AddSub3/1, AddSub1/1
  twiddle/1(a_re) -> AddSub2/1, AddSub/1
  sync/1 -> twiddle/3(sync)
  b/1 -> twiddle/2(b)
  a/1 -> twiddle/1(a)
  ri_to_c/1 -> a+bw/1
  ri_to_c1/1 -> a-bw/1
  Delay/1 -> sync_out/1
  AddSub/1 -> Mux/2, Scale/1
  shift/1 -> Delay3/1
  Scale/1 -> Mux/3
  Delay3/1 -> Mux3/1, Mux2/1, Mux1/1, Mux/1
  Logical/1 -> of/1
  twiddle/5(sync_out) -> Delay/1

== system fft_test/fft/fft_biplex0/biplex_core/fft_stage_3/delay_b ==
  In1 : Inport  OutDataType=sfix(16)  OutScaling=2^0
  delay_slr : xbsIndex_r4/Delay  en=off  latency=DelayLen  dbl_ovrd=off  reg_retiming=off  block_type=delay
      settings: xl_area=[0, 0, 0, 0, 0, 0, 0]  block_version=9.1.01
  Out1 : Outport  OutDataType=sfix(16)  OutScaling=2^0
  wires:
  delay_slr/1 -> Out1/1
  In1/1 -> delay_slr/1

== system fft_test/fft/fft_biplex0/biplex_core/fft_stage_3/delay_f ==
  In1 : Inport  OutDataType=sfix(16)  OutScaling=2^0
  delay_slr : xbsIndex_r4/Delay  en=off  latency=DelayLen  dbl_ovrd=off  reg_retiming=off  block_type=delay
      settings: xl_area=[0, 0, 0, 0, 0, 0, 0]  block_version=9.1.01
  Out1 : Outport  OutDataType=sfix(16)  OutScaling=2^0
  wires:
  delay_slr/1 -> Out1/1
  In1/1 -> delay_slr/1

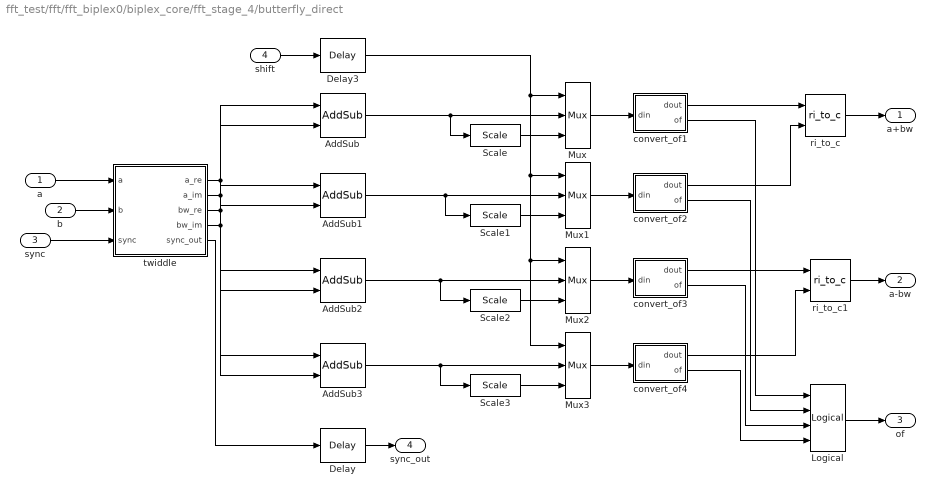
== system fft_test/fft/fft_biplex0/biplex_core/fft_stage_4/butterfly_direct ==
  a : Inport  OutDataType=sfix(16)  OutScaling=2^0
  b : Inport  Port=2  OutDataType=sfix(16)  OutScaling=2^0
  sync : Inport  Port=3  OutDataType=sfix(16)  OutScaling=2^0
  shift : Inport  Port=4  OutDataType=sfix(16)  OutScaling=2^0
  AddSub : xbsIndex_r4/AddSub  mode=Addition  use_carryin=off  use_carryout=off  en=off  latency=add_latency  precision=Full  arith_type=Unsigned  n_bits=8  bin_pt=2  quantization=Truncate  overflow=Wrap  dbl_ovrd=off  use_behavioral_HDL=off  hw_selection=DSP48  pipelined=on  use_rpm=on  block_type=addsub
      settings: xl_area=[0, 0, 0, 0, 0, 0, 0]  block_version=9.1.01
  AddSub1 : xbsIndex_r4/AddSub  mode=Addition  use_carryin=off  use_carryout=off  en=off  latency=add_latency  precision=Full  arith_type=Unsigned  n_bits=8  bin_pt=2  quantization=Truncate  overflow=Wrap  dbl_ovrd=off  use_behavioral_HDL=off  hw_selection=DSP48  pipelined=on  use_rpm=on  block_type=addsub
      settings: xl_area=[0, 0, 0, 0, 0, 0, 0]  block_version=9.1.01
  AddSub2 : xbsIndex_r4/AddSub  mode=Subtraction  use_carryin=off  use_carryout=off  en=off  latency=add_latency  precision=Full  arith_type=Unsigned  n_bits=8  bin_pt=2  quantization=Truncate  overflow=Wrap  dbl_ovrd=off  use_behavioral_HDL=off  hw_selection=DSP48  pipelined=on  use_rpm=on  block_type=addsub
      settings: xl_area=[0, 0, 0, 0, 0, 0, 0]  block_version=9.1.01
  AddSub3 : xbsIndex_r4/AddSub  mode=Subtraction  use_carryin=off  use_carryout=off  en=off  latency=add_latency  precision=Full  arith_type=Unsigned  n_bits=8  bin_pt=2  quantization=Truncate  overflow=Wrap  dbl_ovrd=off  use_behavioral_HDL=off  hw_selection=DSP48  pipelined=on  use_rpm=on  block_type=addsub
      settings: xl_area=[0, 0, 0, 0, 0, 0, 0]  block_version=9.1.01
  Delay : xbsIndex_r4/Delay  en=off  latency=add_latency + conv_latency + 1  dbl_ovrd=off  reg_retiming=on  block_type=delay
      settings: xl_area=[0, 0, 0, 0, 0, 0, 0]  block_version=9.1.01
  Delay3 : xbsIndex_r4/Delay  en=off  latency=add_latency  dbl_ovrd=off  reg_retiming=off  block_type=delay
      settings: xl_area=[0, 0, 0, 0, 0, 0, 0]  block_version=9.1.01
  Logical : xbsIndex_r4/Logical  logical_function=OR  inputs=4  en=off  latency=0  precision=Full  arith_type=Unsigned  n_bits=16  bin_pt=0  align_bp=on  dbl_ovrd=off  block_type=logical
      settings: block_version=10.1.1
  Mux{,1..3} (4 alike) : xbsIndex_r4/Mux  inputs=2  en=off  latency=1  precision=Full  arith_type="Signed  (2's comp)"  n_bits=8  bin_pt=2  quantization=Truncate  overflow=Wrap  dbl_ovrd=off  block_type=mux
      settings: xl_area=[0, 0, 0, 0, 0, 0, 0]  block_version=9.1.01
  Scale{,1..3} (4 alike) : xbsIndex_r4/Scale  scale_factor=-1  dbl_ovrd=off  block_type=scale
      settings: infoedit=Scales input by a power of two by adjusting the binary point position.<P><P>Hardware notes: In hardware this block costs nothing.  block_version=9.1.01
  convert_of1 : Subsystem  AncestorBlock=casper_library_misc/convert_of  mask(convert_of){bit_width_i=15, binary_point_i=10, bit_width_o=8, binary_point_o=7, latency=2, overflow=Saturate, quantization=Round  (unbiased: +/- Inf)}
      mask prompts: bit_width_i "Bit Width In"; binary_point_i "Binary Point In"; bit_width_o "Bit Width Out"; binary_point_o "Binary Point Out"; overflow "Overflow Behaviour"; quantization "Quantization Behaviour"
      mask help:
      | Converts from one 2's complement bit-width
      | and/or binary point position to another.
      | Includes underflow/overflow indicator.
      mask init: same as fft_test/fft/fft_direct/butterfly1_0/convert_of1
      settings: AttributesFormatString=[15,10]->[8,7]
      mask StyleString: edit,edit,edit,edit,edit,popup(Wrap|Saturate|Error),popup(Truncate|Round  (unbiased: +/- Inf)|Round  (unbiased: even values))
  convert_of2 : Subsystem  AncestorBlock=casper_library_misc/convert_of  mask(convert_of){bit_width_i=15, binary_point_i=10, bit_width_o=8, binary_point_o=7, latency=2, overflow=Saturate, quantization=Round  (unbiased: +/- Inf)}
      mask prompts: bit_width_i "Bit Width In"; binary_point_i "Binary Point In"; bit_width_o "Bit Width Out"; binary_point_o "Binary Point Out"; overflow "Overflow Behaviour"; quantization "Quantization Behaviour"
      mask help:
      | Converts from one 2's complement bit-width
      | and/or binary point position to another.
      | Includes underflow/overflow indicator.
      mask init: same as fft_test/fft/fft_direct/butterfly1_0/convert_of1
      settings: AttributesFormatString=[15,10]->[8,7]
      mask StyleString: edit,edit,edit,edit,edit,popup(Wrap|Saturate|Error),popup(Truncate|Round  (unbiased: +/- Inf)|Round  (unbiased: even values))
  convert_of3 : Subsystem  AncestorBlock=casper_library_misc/convert_of  mask(convert_of){bit_width_i=15, binary_point_i=10, bit_width_o=8, binary_point_o=7, latency=2, overflow=Saturate, quantization=Round  (unbiased: +/- Inf)}
      mask prompts: bit_width_i "Bit Width In"; binary_point_i "Binary Point In"; bit_width_o "Bit Width Out"; binary_point_o "Binary Point Out"; overflow "Overflow Behaviour"; quantization "Quantization Behaviour"
      mask help:
      | Converts from one 2's complement bit-width
      | and/or binary point position to another.
      | Includes underflow/overflow indicator.
      mask init: same as fft_test/fft/fft_direct/butterfly1_0/convert_of1
      settings: AttributesFormatString=[15,10]->[8,7]
      mask StyleString: edit,edit,edit,edit,edit,popup(Wrap|Saturate|Error),popup(Truncate|Round  (unbiased: +/- Inf)|Round  (unbiased: even values))
  convert_of4 : Subsystem  AncestorBlock=casper_library_misc/convert_of  mask(convert_of){bit_width_i=15, binary_point_i=10, bit_width_o=8, binary_point_o=7, latency=2, overflow=Saturate, quantization=Round  (unbiased: +/- Inf)}
      mask prompts: bit_width_i "Bit Width In"; binary_point_i "Binary Point In"; bit_width_o "Bit Width Out"; binary_point_o "Binary Point Out"; overflow "Overflow Behaviour"; quantization "Quantization Behaviour"
      mask help:
      | Converts from one 2's complement bit-width
      | and/or binary point position to another.
      | Includes underflow/overflow indicator.
      mask init: same as fft_test/fft/fft_direct/butterfly1_0/convert_of1
      settings: AttributesFormatString=[15,10]->[8,7]
      mask StyleString: edit,edit,edit,edit,edit,popup(Wrap|Saturate|Error),popup(Truncate|Round  (unbiased: +/- Inf)|Round  (unbiased: even values))
  ri_to_c : casper_library_misc/ri_to_c  SystemSampleTime=-1
  ri_to_c1 : casper_library_misc/ri_to_c  SystemSampleTime=-1
  twiddle : Subsystem  AncestorBlock=casper_library_ffts_twiddle/twiddle_general_3mult  mask(twiddle_general_3mult){Coeffs=getfield( getfield( get_param( gcb,'UserData' ), 'parameters'),'Coeffs'), StepPeriod=0, coeffs_bram=off, coeff_bit_width=8, input_bit_width=8, add_latency=2, mult_latency=3, bram_latency=1, conv_latency=2, arch=Virtex5, use_hdl=on, use_embedded=off, quantization=Round  (unbiased: +/- Inf), overflow=Saturate}
      mask prompts: Coeffs "Coefficients:"; StepPeriod "Coefficient Step Period (2^?)"; coeffs_bram "Store coefficients in BRAM"; coeff_bit_width "Coefficient Bit Width"; input_bit_width "Input Bit Width"; add_latency "Add Latency"; mult_latency "Mult Latency"; bram_latency "BRAM Latency"; conv_latency "Convert latency"; arch "Architecture"; use_hdl "Use behavioral HDL for multlipliers"; use_embedded "Use embedded multipliers"; quantization "Quantization Behavior"; overflow "Overflow Behavior"
      mask help:
      | Used in biplex pipelined FFT. Takes advantage that
      | (a+bi)(c+di)=(c(a+b)-b(c+d))+i(b(c+d)+a(c-d)) to
      | save on multipliers at expense of adders.
      mask init: same as fft_test/fft/fft_direct/butterfly1_0/twiddle
      settings: AttributesFormatString=|
      | data=(8,7)
      | coeffs=(7,5)
      | Virtex5
      | (Round  (unbiased: +/- Inf),Saturate)
      mask StyleString: edit,edit,checkbox,edit,edit,edit,edit,edit,edit,popup(Virtex2Pro|Virtex5),checkbox,checkbox,popup(Truncate|Round  (unbiased: +/- Inf)|Round  (unbiased: Even Values)),popup(Wrap|Saturate|Error)
      mask CallbackString:
      | ||||||||||use_hdl = get_param(gcb,'use_hdl');
      | visibs = get_param(gcb, 'MaskVisibilities');
      | if( strcmp(use_hdl,'on')),
      |     set_param(gcb, 'use_embedded','off');
      |     visibs{12} = 'off';
      | else,
      |     visibs{12} = 'on';
      | end
      | set_param(gcb, 'MaskVisibilities', visibs);
      | |||
  a+bw : Outport  OutDataType=sfix(16)  OutScaling=2^0
  a-bw : Outport  Port=2  OutDataType=sfix(16)  OutScaling=2^0
  of : Outport  Port=3  OutDataType=sfix(16)  OutScaling=2^0
  sync_out : Outport  Port=4  OutDataType=sfix(16)  OutScaling=2^0
  wires:
  convert_of4/2(of) -> Logical/4
  convert_of3/2(of) -> Logical/3
  convert_of2/2(of) -> Logical/2
  convert_of1/2(of) -> Logical/1
  convert_of4/1(dout) -> ri_to_c1/2
  Mux3/1 -> convert_of4/1(din)
  AddSub3/1 -> Scale3/1, Mux3/2
  Scale3/1 -> Mux3/3
  convert_of3/1(dout) -> ri_to_c1/1
  Mux2/1 -> convert_of3/1(din)
  AddSub2/1 -> Scale2/1, Mux2/2
  Scale2/1 -> Mux2/3
  convert_of2/1(dout) -> ri_to_c/2
  Mux1/1 -> convert_of2/1(din)
  AddSub1/1 -> Scale1/1, Mux1/2
  Scale1/1 -> Mux1/3
  convert_of1/1(dout) -> ri_to_c/1
  Mux/1 -> convert_of1/1(din)
  twiddle/4(bw_im) -> AddSub3/2, AddSub1/2
  twiddle/3(bw_re) -> AddSub2/2, AddSub/2
  twiddle/2(a_im) -> AddSub3/1, AddSub1/1
  twiddle/1(a_re) -> AddSub2/1, AddSub/1
  sync/1 -> twiddle/3(sync)
  b/1 -> twiddle/2(b)
  a/1 -> twiddle/1(a)
  ri_to_c/1 -> a+bw/1
  ri_to_c1/1 -> a-bw/1
  Delay/1 -> sync_out/1
  AddSub/1 -> Mux/2, Scale/1
  shift/1 -> Delay3/1
  Scale/1 -> Mux/3
  Delay3/1 -> Mux3/1, Mux2/1, Mux1/1, Mux/1
  Logical/1 -> of/1
  twiddle/5(sync_out) -> Delay/1

== system fft_test/fft/fft_biplex0/biplex_core/fft_stage_4/delay_b ==
  In1 : Inport  OutDataType=sfix(16)  OutScaling=2^0
  delay_slr : xbsIndex_r4/Delay  en=off  latency=DelayLen  dbl_ovrd=off  reg_retiming=off  block_type=delay
      settings: xl_area=[0, 0, 0, 0, 0, 0, 0]  block_version=9.1.01
  Out1 : Outport  OutDataType=sfix(16)  OutScaling=2^0
  wires:
  delay_slr/1 -> Out1/1
  In1/1 -> delay_slr/1
